simulink model "orig_exp_linear"  (R2023a)
settings: Solver=ode4  StartTime=0.0  StopTime=10  FixedStep=0.001  RelTol=1e-3
settings Model: Creator=Anonymous  LastModifiedBy=Anonymous

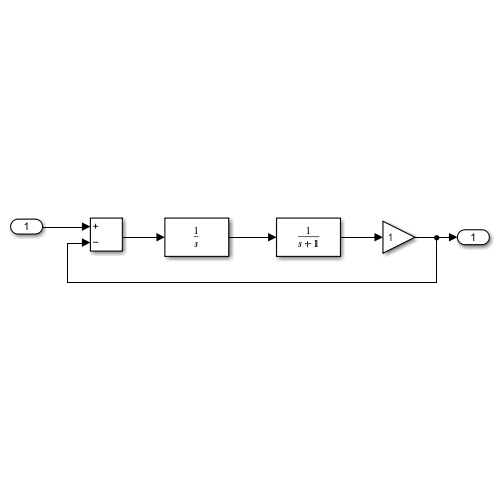
[thumbnail: Simulink's stored preview of the top-level diagram]
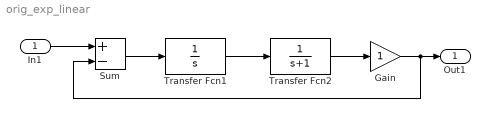
== system orig_exp_linear ==
  In1 : Inport
  Gain : Gain
  Sum : Sum  Inputs=+-
  Transfer Fcn1 : TransferFcn  Numerator=1  Denominator=[1 0]
  Transfer Fcn2 : TransferFcn  Numerator=1  Denominator=[1 1]
  Out1 : Outport
  wires:
  Gain/1 -> Sum/2, Out1/1
  Transfer Fcn2/1 -> Gain/1
  Transfer Fcn1/1 -> Transfer Fcn2/1
  Sum/1 -> Transfer Fcn1/1
  In1/1 -> Sum/1
